simulink model "MotorFaultDeploy"  (R2026a)
settings: Solver=FixedStepDiscrete  FixedStep=1/12000
settings Model: Creator=Tejashri  LastModifiedBy=Tejashri
settings HardwareCC: ProdLargestAtomicInteger=Long  ProdLargestAtomicFloat=Double  ProdHWDeviceType=ARM Compatible->ARM Cortex-M
settings RTWCC: GenCodeOnly=on  GenerateReport=on

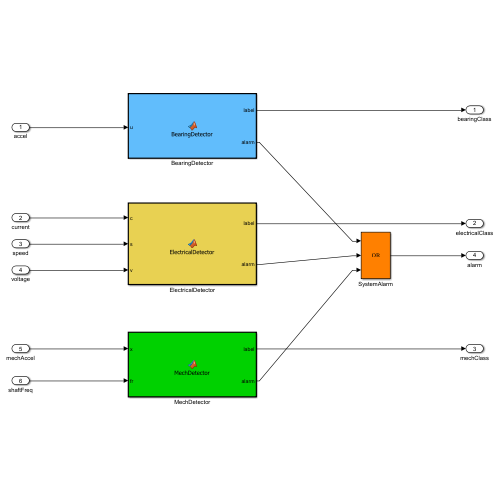
[thumbnail: Simulink's stored preview of the top-level diagram]
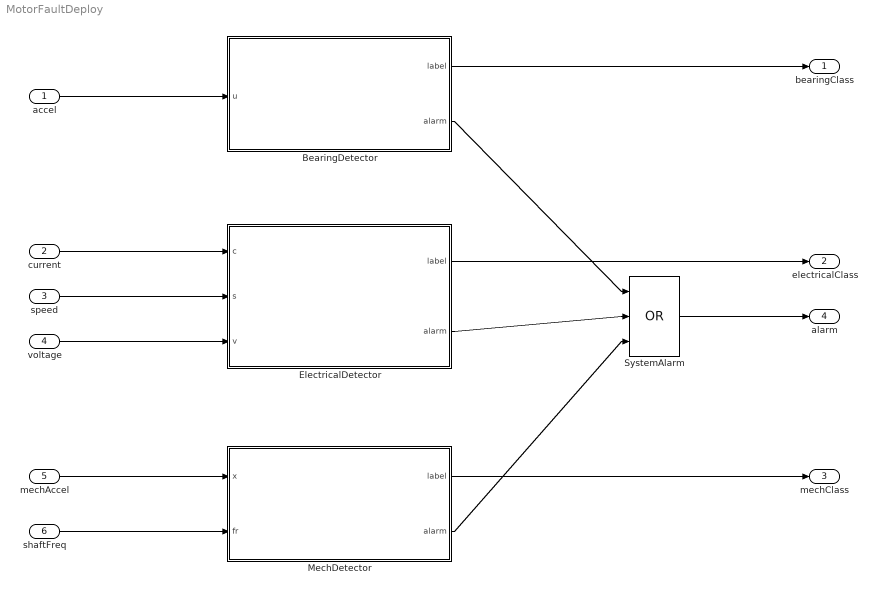
== system MotorFaultDeploy ==
  accel : Inport  SampleTime=1/12000
  current : Inport  Port=2  SampleTime=1/12000
  speed : Inport  Port=3  SampleTime=1/12000
  voltage : Inport  Port=4  SampleTime=1/12000
  mechAccel : Inport  Port=5  SampleTime=1/12000
  shaftFreq : Inport  Port=6  SampleTime=1/12000
  BearingDetector : MATLAB Function  TreatAsAtomicUnit=on
  ElectricalDetector : MATLAB Function  TreatAsAtomicUnit=on
  MechDetector : MATLAB Function  TreatAsAtomicUnit=on
  SystemAlarm : Logic  Operator=OR  Inputs=3  AllPortsSameDT=off  OutDataTypeStr=boolean
  bearingClass : Outport
  electricalClass : Outport  Port=2
  mechClass : Outport  Port=3
  alarm : Outport  Port=4
  wires:
  accel/1 -> BearingDetector/1(u)
  current/1 -> ElectricalDetector/1(c)
  speed/1 -> ElectricalDetector/2(s)
  voltage/1 -> ElectricalDetector/3(v)
  mechAccel/1 -> MechDetector/1(x)
  shaftFreq/1 -> MechDetector/2(fr)
  BearingDetector/2(alarm) -> SystemAlarm/1
  ElectricalDetector/2(alarm) -> SystemAlarm/2
  MechDetector/2(alarm) -> SystemAlarm/3
  BearingDetector/1(label) -> bearingClass/1
  ElectricalDetector/1(label) -> electricalClass/1
  MechDetector/1(label) -> mechClass/1
  SystemAlarm/1 -> alarm/1

== matlab function MotorFaultDeploy/ElectricalDetector ==
  data: c input; label output; s input; v input; alarm output
function [label, alarm] = ElectricalDetector(c, s, v)
[label, alarm] = electricalDetector(c, s, v);

== matlab function MotorFaultDeploy/BearingDetector ==
  data: u input; label output; alarm output
function [label, alarm] = BearingDetector(u)
[label, alarm] = motorDetector(u);

== matlab function MotorFaultDeploy/MechDetector ==
  data: x input; label output; fr input; alarm output
function [label, alarm] = MechDetector(x, fr)
[label, alarm] = mechanicalDetector(x, fr);
